simulink model "signal_based_model"  (R2025b)
settings: Solver=VariableStepAuto  StartTime=0.0  StopTime=10  RelTol=1e-3
libraries: slpidlib x4
settings Model: Creator=leo  LastModifiedBy=leo

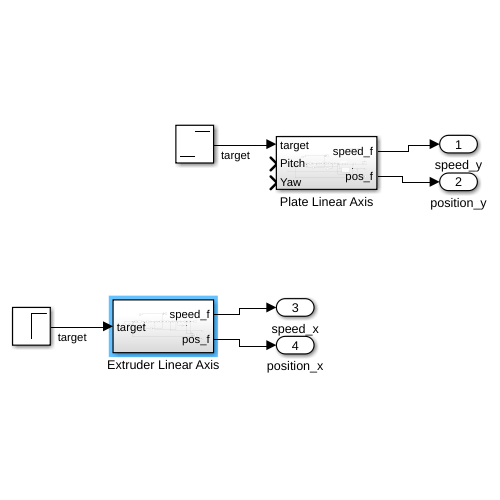
[thumbnail: Simulink's stored preview of the top-level diagram]
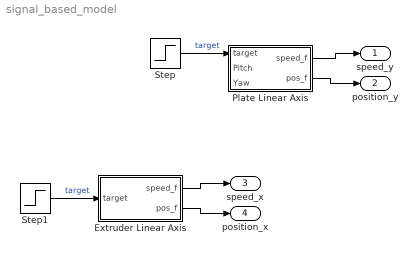
== system signal_based_model ==
  Extruder Linear Axis : Subsystem
  Plate Linear Axis : Subsystem
  Step : Step  After=0.3  SampleTime=0
  Step1 : Step  Time=0  After=0.1  SampleTime=0
  speed_y : Outport
  position_y : Outport  Port=2
  speed_x : Outport  Port=3
  position_x : Outport  Port=4
  wires:
  Step/1 -> Plate Linear Axis/1(target)  "target"
  Plate Linear Axis/1(speed_f) -> speed_y/1
  Extruder Linear Axis/2(pos_f) -> position_x/1
  Extruder Linear Axis/1(speed_f) -> speed_x/1
  Step1/1 -> Extruder Linear Axis/1(target)  "target"
  Plate Linear Axis/2(pos_f) -> position_y/1

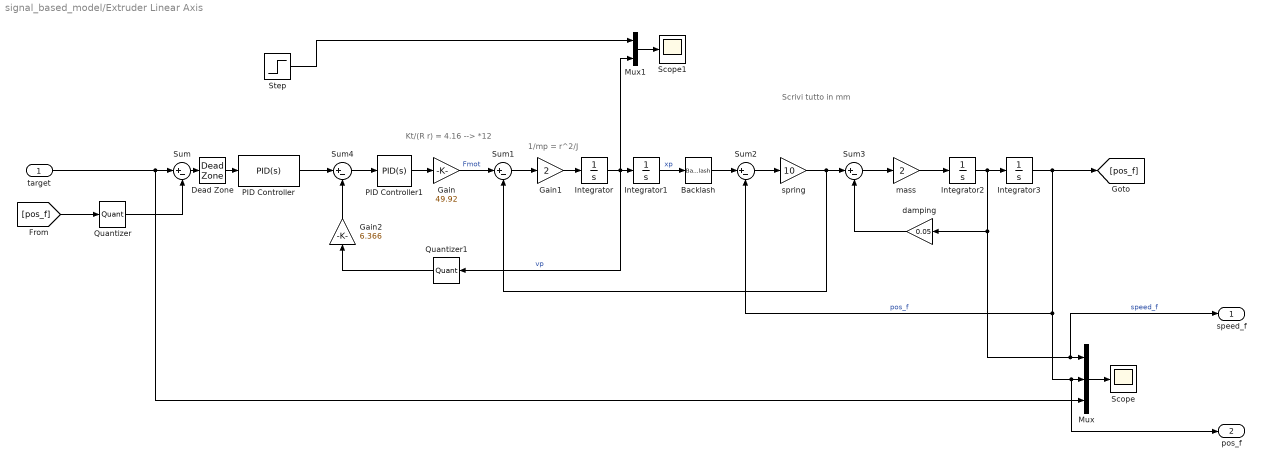
== system signal_based_model/Extruder Linear Axis ==
  note: Scrivi tutto in mm
  note: 1/mp = r^2/J
  note: Kt/(R r) = 4.16 --> *12
  target : Inport
  Backlash : Backlash  BacklashWidth=0.01
  Dead Zone : DeadZone  LowerValue=-0.005  UpperValue=0.005
  Gain : Gain  Gain=49.92
  Gain1 : Gain  Gain=2
  Gain2 : Gain  Gain=6.366
  Integrator{,1..3} (4 alike) : Integrator
  Mux : Mux  Inputs=3
  Mux1 : Mux  Inputs=2
  PID Controller : slpidlib/PID Controller  Controller=PID  Form=Parallel  TimeDomain=Continuous-time  UseExternalTs=off  SampleTime=-1  IntegratorMethod=Forward Euler  FilterMethod=Forward Euler  ControllerParametersSource=internal  P=5.88101312696394  I=1.22832421869703  UseKiTs=off  D=-1.679348597049  UseExternalDerivativeSource=off  N=2.27817359459084  UseFilter=on  TunerSelectOption=Transfer Function Based (PID Tuner App)  InitialConditionSource=internal  InitialConditionForIntegrator=0  InitialConditionForFilter=0  DifferentiatorICPrevScaledInput=0  ExternalReset=none  TrackingMode=off  Kt=1  LimitOutput=on  SatLimitsSource=internal  UpperSaturationLimit=300  LowerSaturationLimit=-300  LinearizeAsGain=on  AntiWindupMode=none  Kb=1  LimitIntegrator=off  UpperIntegratorSaturationLimit=inf  LowerIntegratorSaturationLimit=-inf  POutMin=[]  POutMax=[]  IOutMin=[]  IOutMax=[]  DOutMin=[]  DOutMax=[]  NOutMin=[]  NOutMax=[]  SumOutMin=[]  SumOutMax=[]  SaturationOutMin=[]  SaturationOutMax=[]  PParamMin=[]  PParamMax=[]  IParamMin=[]  IParamMax=[]  DParamMin=[]  DParamMax=[]  NParamMin=[]  NParamMax=[]  KbParamMin=[]  KbParamMax=[]  KtParamMin=[]  KtParamMax=[]  KbOutMin=[]  KbOutMax=[]  KtOutMin=[]  KtOutMax=[]  IntegratorOutMin=[]  IntegratorOutMax=[]  FilterOutMin=[]  FilterOutMax=[]  SumI1OutMin=[]  SumI1OutMax=[]  SumI2OutMin=[]  SumI2OutMax=[]  SumI3OutMin=[]  SumI3OutMax=[]  SumI4OutMin=[]  SumI4OutMax=[]  SumDOutMin=[]  SumDOutMax=[]  DifferentiatorOutMin=[]  DifferentiatorOutMax=[]  FilterDiffOutCoefMin=[]  FilterDiffOutCoefMax=[]  ReciprocalOutMin=[]  ReciprocalOutMax=[]  SumDenOutMin=[]  SumDenOutMax=[]  SumNumOutMin=[]  SumNumOutMax=[]  DivideOutMin=[]  DivideOutMax=[]  UdiffTsProdOutMin=[]  UdiffTsProdOutMax=[]  NTsProdOutMin=[]  NTsProdOutMax=[]  UintegralTsProdOutMin=[]  UintegralTsProdOutMax=[]  UngainTsProdOutMin=[]  UngainTsProdOutMax=[]  ClampingZeroOutDataTypeStr=Inherit: Inherit via back propagation  ClampingZeroOutMin=[]  ClampingZeroOutMax=[]  FilterDenConstantOutDataTypeStr=Inherit: Inherit via back propagation  FilterDenConstantOutMin=[]  FilterDenConstantOutMax=[]  PCopyOutDataTypeStr=Inherit: Inherit via back propagation  PCopyOutMin=[]  PCopyOutMax=[]  NCopyOutDataTypeStr=Inherit: Inherit via back propagation  NCopyOutMin=[]  NCopyOutMax=[]  IntegratorContinuousStateAttributes=''  IntegratorStateMustResolveToSignalObject=off  IntegratorRTWStateStorageClass=Auto  FilterContinuousStateAttributes=''  FilterStateMustResolveToSignalObject=off  FilterRTWStateStorageClass=Auto  ParallelPVariant=InternalParameters  IdealPVariant=Disabled  IVariant=InternalParameters  DVariant=InternalParameters  IntegratorVariant=Continuous  SatVariant=Enabled  AWVariant=Passthrough  PCopyVariant=Disabled  TRVariant=Disabled  FdbkBlocksVariant=Forward  IdealPFdbkVariant=Disabled  SatFdbkVariant=Disabled  DerivativeFilterVariant=ContFilter  NVariant=InternalParameters  NCopyVariant=Disabled  FilterICVariant=InternalICsFilter  IntegratorICVariant=InternalICs  ExternalResetVariant=Disabled  TRSumVariant=Passthrough  SumFdbkVariant=Disabled  SumVariant=Sum_PID  TsampFilterVariant=InternalTs  TsampNgainVariant=Passthrough  TsampIntegralVariant=Disabled_SignalSpec  ExternalSaturationOutDataTypeStr=Inherit: Same as second input  DerivativeSourceVariant=ErrorSignal  PreIntVariant=InternalPreInt
  PID Controller1 : slpidlib/PID Controller  Controller=PID  Form=Parallel  TimeDomain=Continuous-time  UseExternalTs=off  SampleTime=-1  IntegratorMethod=Forward Euler  FilterMethod=Forward Euler  ControllerParametersSource=internal  P=0.0150067865506817  I=0.0265065175500297  UseKiTs=off  D=0.000284995898305726  UseExternalDerivativeSource=off  N=36.46824066771  UseFilter=on  TunerSelectOption=Transfer Function Based (PID Tuner App)  InitialConditionSource=internal  InitialConditionForIntegrator=0  InitialConditionForFilter=0  DifferentiatorICPrevScaledInput=0  ExternalReset=none  TrackingMode=off  Kt=1  LimitOutput=on  SatLimitsSource=internal  UpperSaturationLimit=1  LowerSaturationLimit=-1  LinearizeAsGain=on  AntiWindupMode=none  Kb=1  LimitIntegrator=off  UpperIntegratorSaturationLimit=inf  LowerIntegratorSaturationLimit=-inf  POutMin=[]  POutMax=[]  IOutMin=[]  IOutMax=[]  DOutMin=[]  DOutMax=[]  NOutMin=[]  NOutMax=[]  SumOutMin=[]  SumOutMax=[]  SaturationOutMin=[]  SaturationOutMax=[]  PParamMin=[]  PParamMax=[]  IParamMin=[]  IParamMax=[]  DParamMin=[]  DParamMax=[]  NParamMin=[]  NParamMax=[]  KbParamMin=[]  KbParamMax=[]  KtParamMin=[]  KtParamMax=[]  KbOutMin=[]  KbOutMax=[]  KtOutMin=[]  KtOutMax=[]  IntegratorOutMin=[]  IntegratorOutMax=[]  FilterOutMin=[]  FilterOutMax=[]  SumI1OutMin=[]  SumI1OutMax=[]  SumI2OutMin=[]  SumI2OutMax=[]  SumI3OutMin=[]  SumI3OutMax=[]  SumI4OutMin=[]  SumI4OutMax=[]  SumDOutMin=[]  SumDOutMax=[]  DifferentiatorOutMin=[]  DifferentiatorOutMax=[]  FilterDiffOutCoefMin=[]  FilterDiffOutCoefMax=[]  ReciprocalOutMin=[]  ReciprocalOutMax=[]  SumDenOutMin=[]  SumDenOutMax=[]  SumNumOutMin=[]  SumNumOutMax=[]  DivideOutMin=[]  DivideOutMax=[]  UdiffTsProdOutMin=[]  UdiffTsProdOutMax=[]  NTsProdOutMin=[]  NTsProdOutMax=[]  UintegralTsProdOutMin=[]  UintegralTsProdOutMax=[]  UngainTsProdOutMin=[]  UngainTsProdOutMax=[]  ClampingZeroOutDataTypeStr=Inherit: Inherit via back propagation  ClampingZeroOutMin=[]  ClampingZeroOutMax=[]  FilterDenConstantOutDataTypeStr=Inherit: Inherit via back propagation  FilterDenConstantOutMin=[]  FilterDenConstantOutMax=[]  PCopyOutDataTypeStr=Inherit: Inherit via back propagation  PCopyOutMin=[]  PCopyOutMax=[]  NCopyOutDataTypeStr=Inherit: Inherit via back propagation  NCopyOutMin=[]  NCopyOutMax=[]  IntegratorContinuousStateAttributes=''  IntegratorStateMustResolveToSignalObject=off  IntegratorRTWStateStorageClass=Auto  FilterContinuousStateAttributes=''  FilterStateMustResolveToSignalObject=off  FilterRTWStateStorageClass=Auto  ParallelPVariant=InternalParameters  IdealPVariant=Disabled  IVariant=InternalParameters  DVariant=InternalParameters  IntegratorVariant=Continuous  SatVariant=Enabled  AWVariant=Passthrough  PCopyVariant=Disabled  TRVariant=Disabled  FdbkBlocksVariant=Forward  IdealPFdbkVariant=Disabled  SatFdbkVariant=Disabled  DerivativeFilterVariant=ContFilter  NVariant=InternalParameters  NCopyVariant=Disabled  FilterICVariant=InternalICsFilter  IntegratorICVariant=InternalICs  ExternalResetVariant=Disabled  TRSumVariant=Passthrough  SumFdbkVariant=Disabled  SumVariant=Sum_PID  TsampFilterVariant=InternalTs  TsampNgainVariant=Passthrough  TsampIntegralVariant=Disabled_SignalSpec  ExternalSaturationOutDataTypeStr=Inherit: Same as second input  DerivativeSourceVariant=ErrorSignal  PreIntVariant=InternalPreInt
  Quantizer : Quantizer  QuantizationInterval=0.005
  Quantizer1 : Quantizer  QuantizationInterval=0.02
  Scope : Scope
      settings: ActiveDisplayYMinimum=-0.12448091538103732  ActiveDisplayYMaximum=0.19087454091258427
  Scope1 : Scope
      settings: ActiveDisplayYMinimum=-1  ActiveDisplayYMaximum=1
  Step : Step  After=250  SampleTime=0
  Sum{,1..4} (5 alike) : Sum  Inputs=|+-
  damping : Gain  Gain=0.05
  mass : Gain  Gain=2
  spring : Gain  Gain=10
  speed_f : Outport
  pos_f : Outport  Port=2
  wires:
  Integrator/1 -> Mux1/2, Quantizer1/1, Integrator1/1  "vp"
  Integrator1/1 -> Backlash/1  "xp"
  Integrator3/1 -> [pos_f], Sum2/2, pos_f/1, Mux/2  "pos_f"
  Integrator2/1 -> speed_f/1, Mux/1, damping/1, Integrator3/1  "speed_f"
  Gain/1 -> Sum1/1  "Fmot"
  Gain1/1 -> Integrator/1
  Sum3/1 -> mass/1
  damping/1 -> Sum3/2
  spring/1 -> Sum1/2, Sum3/1
  Mux/1 -> Scope/1
  Sum1/1 -> Gain1/1
  Sum2/1 -> spring/1
  mass/1 -> Integrator2/1
  target/1 -> Mux/3, Sum/1
  [pos_f] -> Quantizer/1
  Backlash/1 -> Sum2/1
  Sum/1 -> Dead Zone/1
  Dead Zone/1 -> PID Controller/1
  PID Controller1/1 -> Gain/1
  Sum4/1 -> PID Controller1/1
  Quantizer1/1 -> Gain2/1
  Step/1 -> Mux1/1
  Mux1/1 -> Scope1/1
  Quantizer/1 -> Sum/2
  Gain2/1 -> Sum4/2
  PID Controller/1 -> Sum4/1

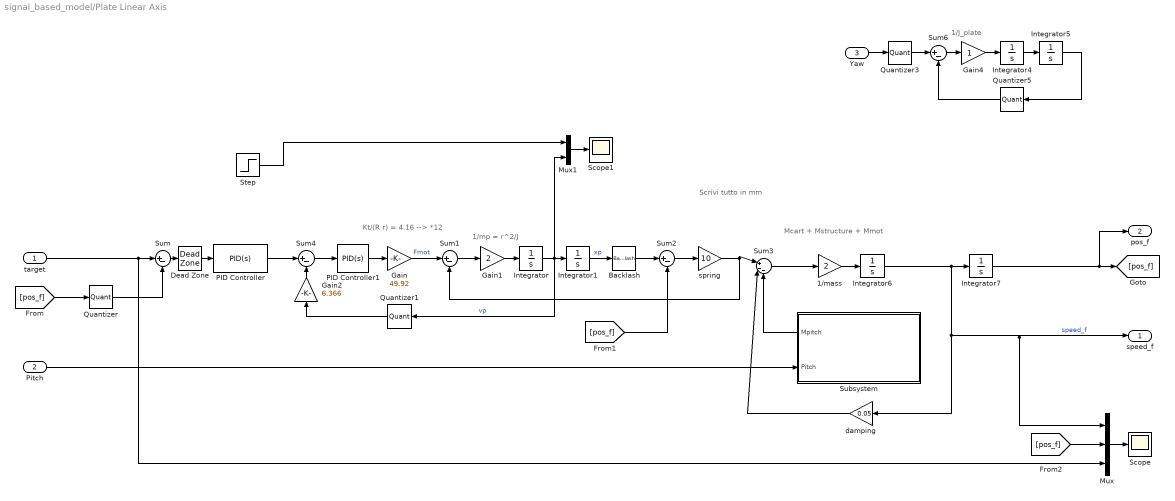
== system signal_based_model/Plate Linear Axis ==
  note: Scrivi tutto in mm
  note: 1/mp = r^2/J
  note: Kt/(R r) = 4.16 --> *12
  note: 1/J_plate
  note: Mcart + Mstructure + Mmot
  target : Inport
  Pitch : Inport  Port=2
  Yaw : Inport  Port=3
  1/mass : Gain  Gain=2
  Backlash : Backlash  BacklashWidth=0.01
  Dead Zone : DeadZone  LowerValue=-0.005  UpperValue=0.005
  Gain : Gain  Gain=49.92
  Gain1 : Gain  Gain=2
  Gain2 : Gain  Gain=6.366
  Gain4 : Gain
  Integrator{,1,4..7} (6 alike) : Integrator
  Mux : Mux  Inputs=3
  Mux1 : Mux  Inputs=2
  PID Controller : slpidlib/PID Controller  Controller=PID  Form=Parallel  TimeDomain=Continuous-time  UseExternalTs=off  SampleTime=-1  IntegratorMethod=Forward Euler  FilterMethod=Forward Euler  ControllerParametersSource=internal  P=3.73662295792307  I=0.466470585672945  UseKiTs=off  D=-1.58456449848514  UseExternalDerivativeSource=off  N=2.35813875768094  UseFilter=on  TunerSelectOption=Transfer Function Based (PID Tuner App)  InitialConditionSource=internal  InitialConditionForIntegrator=0  InitialConditionForFilter=0  DifferentiatorICPrevScaledInput=0  ExternalReset=none  TrackingMode=off  Kt=1  LimitOutput=on  SatLimitsSource=internal  UpperSaturationLimit=300  LowerSaturationLimit=-300  LinearizeAsGain=on  AntiWindupMode=none  Kb=1  LimitIntegrator=off  UpperIntegratorSaturationLimit=inf  LowerIntegratorSaturationLimit=-inf  POutMin=[]  POutMax=[]  IOutMin=[]  IOutMax=[]  DOutMin=[]  DOutMax=[]  NOutMin=[]  NOutMax=[]  SumOutMin=[]  SumOutMax=[]  SaturationOutMin=[]  SaturationOutMax=[]  PParamMin=[]  PParamMax=[]  IParamMin=[]  IParamMax=[]  DParamMin=[]  DParamMax=[]  NParamMin=[]  NParamMax=[]  KbParamMin=[]  KbParamMax=[]  KtParamMin=[]  KtParamMax=[]  KbOutMin=[]  KbOutMax=[]  KtOutMin=[]  KtOutMax=[]  IntegratorOutMin=[]  IntegratorOutMax=[]  FilterOutMin=[]  FilterOutMax=[]  SumI1OutMin=[]  SumI1OutMax=[]  SumI2OutMin=[]  SumI2OutMax=[]  SumI3OutMin=[]  SumI3OutMax=[]  SumI4OutMin=[]  SumI4OutMax=[]  SumDOutMin=[]  SumDOutMax=[]  DifferentiatorOutMin=[]  DifferentiatorOutMax=[]  FilterDiffOutCoefMin=[]  FilterDiffOutCoefMax=[]  ReciprocalOutMin=[]  ReciprocalOutMax=[]  SumDenOutMin=[]  SumDenOutMax=[]  SumNumOutMin=[]  SumNumOutMax=[]  DivideOutMin=[]  DivideOutMax=[]  UdiffTsProdOutMin=[]  UdiffTsProdOutMax=[]  NTsProdOutMin=[]  NTsProdOutMax=[]  UintegralTsProdOutMin=[]  UintegralTsProdOutMax=[]  UngainTsProdOutMin=[]  UngainTsProdOutMax=[]  ClampingZeroOutDataTypeStr=Inherit: Inherit via back propagation  ClampingZeroOutMin=[]  ClampingZeroOutMax=[]  FilterDenConstantOutDataTypeStr=Inherit: Inherit via back propagation  FilterDenConstantOutMin=[]  FilterDenConstantOutMax=[]  PCopyOutDataTypeStr=Inherit: Inherit via back propagation  PCopyOutMin=[]  PCopyOutMax=[]  NCopyOutDataTypeStr=Inherit: Inherit via back propagation  NCopyOutMin=[]  NCopyOutMax=[]  IntegratorContinuousStateAttributes=''  IntegratorStateMustResolveToSignalObject=off  IntegratorRTWStateStorageClass=Auto  FilterContinuousStateAttributes=''  FilterStateMustResolveToSignalObject=off  FilterRTWStateStorageClass=Auto  ParallelPVariant=InternalParameters  IdealPVariant=Disabled  IVariant=InternalParameters  DVariant=InternalParameters  IntegratorVariant=Continuous  SatVariant=Enabled  AWVariant=Passthrough  PCopyVariant=Disabled  TRVariant=Disabled  FdbkBlocksVariant=Forward  IdealPFdbkVariant=Disabled  SatFdbkVariant=Disabled  DerivativeFilterVariant=ContFilter  NVariant=InternalParameters  NCopyVariant=Disabled  FilterICVariant=InternalICsFilter  IntegratorICVariant=InternalICs  ExternalResetVariant=Disabled  TRSumVariant=Passthrough  SumFdbkVariant=Disabled  SumVariant=Sum_PID  TsampFilterVariant=InternalTs  TsampNgainVariant=Passthrough  TsampIntegralVariant=Disabled_SignalSpec  ExternalSaturationOutDataTypeStr=Inherit: Same as second input  DerivativeSourceVariant=ErrorSignal  PreIntVariant=InternalPreInt
  PID Controller1 : slpidlib/PID Controller  Controller=PID  Form=Parallel  TimeDomain=Continuous-time  UseExternalTs=off  SampleTime=-1  IntegratorMethod=Forward Euler  FilterMethod=Forward Euler  ControllerParametersSource=internal  P=0.0150067865506817  I=0.0265065175500297  UseKiTs=off  D=0.000284995898305726  UseExternalDerivativeSource=off  N=36.46824066771  UseFilter=on  TunerSelectOption=Transfer Function Based (PID Tuner App)  InitialConditionSource=internal  InitialConditionForIntegrator=0  InitialConditionForFilter=0  DifferentiatorICPrevScaledInput=0  ExternalReset=none  TrackingMode=off  Kt=1  LimitOutput=on  SatLimitsSource=internal  UpperSaturationLimit=1  LowerSaturationLimit=-1  LinearizeAsGain=on  AntiWindupMode=none  Kb=1  LimitIntegrator=off  UpperIntegratorSaturationLimit=inf  LowerIntegratorSaturationLimit=-inf  POutMin=[]  POutMax=[]  IOutMin=[]  IOutMax=[]  DOutMin=[]  DOutMax=[]  NOutMin=[]  NOutMax=[]  SumOutMin=[]  SumOutMax=[]  SaturationOutMin=[]  SaturationOutMax=[]  PParamMin=[]  PParamMax=[]  IParamMin=[]  IParamMax=[]  DParamMin=[]  DParamMax=[]  NParamMin=[]  NParamMax=[]  KbParamMin=[]  KbParamMax=[]  KtParamMin=[]  KtParamMax=[]  KbOutMin=[]  KbOutMax=[]  KtOutMin=[]  KtOutMax=[]  IntegratorOutMin=[]  IntegratorOutMax=[]  FilterOutMin=[]  FilterOutMax=[]  SumI1OutMin=[]  SumI1OutMax=[]  SumI2OutMin=[]  SumI2OutMax=[]  SumI3OutMin=[]  SumI3OutMax=[]  SumI4OutMin=[]  SumI4OutMax=[]  SumDOutMin=[]  SumDOutMax=[]  DifferentiatorOutMin=[]  DifferentiatorOutMax=[]  FilterDiffOutCoefMin=[]  FilterDiffOutCoefMax=[]  ReciprocalOutMin=[]  ReciprocalOutMax=[]  SumDenOutMin=[]  SumDenOutMax=[]  SumNumOutMin=[]  SumNumOutMax=[]  DivideOutMin=[]  DivideOutMax=[]  UdiffTsProdOutMin=[]  UdiffTsProdOutMax=[]  NTsProdOutMin=[]  NTsProdOutMax=[]  UintegralTsProdOutMin=[]  UintegralTsProdOutMax=[]  UngainTsProdOutMin=[]  UngainTsProdOutMax=[]  ClampingZeroOutDataTypeStr=Inherit: Inherit via back propagation  ClampingZeroOutMin=[]  ClampingZeroOutMax=[]  FilterDenConstantOutDataTypeStr=Inherit: Inherit via back propagation  FilterDenConstantOutMin=[]  FilterDenConstantOutMax=[]  PCopyOutDataTypeStr=Inherit: Inherit via back propagation  PCopyOutMin=[]  PCopyOutMax=[]  NCopyOutDataTypeStr=Inherit: Inherit via back propagation  NCopyOutMin=[]  NCopyOutMax=[]  IntegratorContinuousStateAttributes=''  IntegratorStateMustResolveToSignalObject=off  IntegratorRTWStateStorageClass=Auto  FilterContinuousStateAttributes=''  FilterStateMustResolveToSignalObject=off  FilterRTWStateStorageClass=Auto  ParallelPVariant=InternalParameters  IdealPVariant=Disabled  IVariant=InternalParameters  DVariant=InternalParameters  IntegratorVariant=Continuous  SatVariant=Enabled  AWVariant=Passthrough  PCopyVariant=Disabled  TRVariant=Disabled  FdbkBlocksVariant=Forward  IdealPFdbkVariant=Disabled  SatFdbkVariant=Disabled  DerivativeFilterVariant=ContFilter  NVariant=InternalParameters  NCopyVariant=Disabled  FilterICVariant=InternalICsFilter  IntegratorICVariant=InternalICs  ExternalResetVariant=Disabled  TRSumVariant=Passthrough  SumFdbkVariant=Disabled  SumVariant=Sum_PID  TsampFilterVariant=InternalTs  TsampNgainVariant=Passthrough  TsampIntegralVariant=Disabled_SignalSpec  ExternalSaturationOutDataTypeStr=Inherit: Same as second input  DerivativeSourceVariant=ErrorSignal  PreIntVariant=InternalPreInt
  Quantizer : Quantizer  QuantizationInterval=0.01
  Quantizer1 : Quantizer  QuantizationInterval=0.02
  Quantizer3 : Quantizer
  Quantizer5 : Quantizer
  Scope : Scope
      settings: ActiveDisplayYMinimum=-1.0744185087165565  ActiveDisplayYMaximum=1.0049223218652417
  Scope1 : Scope
      settings: ActiveDisplayYMinimum=-1  ActiveDisplayYMaximum=1
  Step : Step  After=250  SampleTime=0
  Subsystem : Subsystem
      settings: PortSchema="{\"entries\":[{\"content\":{\"sides\":[{\"content\":{\"connectorIds\":[\"Out1\",\"In1\"]},\"type\":\"ConnectorPlacement.EquallySpacedRectSide\",\"uuid\":\"c6fbe630-3349-497f-9dd7-90e0f83e84b9\"},{\"content\":{\"side\":\"RIGHT\"},\"type\":\"ConnectorPlacement.EquallySpacedRectSide\",\"uuid\":\"ffa0a2d0-f213-47a0-84af-10fed00c1f85\"},{\"content\":{\"side\":\"TOP\"},\"type\":\"ConnectorPlacement.EquallySpacedRectSide\",\"uuid\":\"5dd9fa2b-7a91-4dc9-91b0-f07acfc95730\"}]},\"type\":\"ConnectorPlacement.EquallySpacedConnector\",\"uuid\":\"75913121-a205-499e-a3df-ddb329c0f5be\"}],\"packageUris\":[\"http://schema.mathworks.com/mf0/Connector/R2020b\"],\"version\":\"1.0\"}"
  Sum{,1..2,4,6} (5 alike) : Sum  Inputs=|+-
  Sum3 : Sum  Inputs=|+--
  damping : Gain  Gain=0.05
  spring : Gain  Gain=10
  speed_f : Outport
  pos_f : Outport  Port=2
  wires:
  Integrator/1 -> Mux1/2, Quantizer1/1, Integrator1/1  "vp"
  Integrator1/1 -> Backlash/1  "xp"
  Gain/1 -> Sum1/1  "Fmot"
  Gain1/1 -> Integrator/1
  spring/1 -> Sum1/2, Sum3/1
  Mux/1 -> Scope/1
  Sum1/1 -> Gain1/1
  Sum2/1 -> spring/1
  target/1 -> Mux/3, Sum/1
  [pos_f] -> Quantizer/1
  Backlash/1 -> Sum2/1
  Sum/1 -> Dead Zone/1
  Dead Zone/1 -> PID Controller/1
  PID Controller1/1 -> Gain/1
  Sum4/1 -> PID Controller1/1
  Quantizer1/1 -> Gain2/1
  Step/1 -> Mux1/1
  Mux1/1 -> Scope1/1
  Quantizer/1 -> Sum/2
  Gain2/1 -> Sum4/2
  PID Controller/1 -> Sum4/1
  Integrator7/1 -> pos_f/1, [pos_f]
  Sum3/1 -> 1/mass/1
  Sum6/1 -> Gain4/1
  Quantizer5/1 -> Sum6/2
  Quantizer3/1 -> Sum6/1
  Gain4/1 -> Integrator4/1
  Integrator5/1 -> Quantizer5/1
  Integrator4/1 -> Integrator5/1
  Yaw/1 -> Quantizer3/1
  Integrator6/1 -> damping/1, Mux/1, speed_f/1, Integrator7/1  "speed_f"
  1/mass/1 -> Integrator6/1
  damping/1 -> Sum3/2
  Pitch/1 -> Subsystem/1(Pitch)
  Subsystem/1(Mpitch) -> Sum3/3
  [pos_f] -> Mux/2
  [pos_f] -> Sum2/2

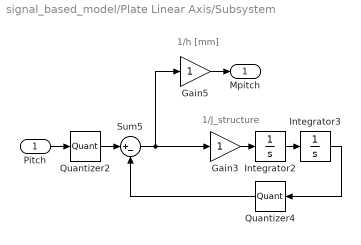
== system signal_based_model/Plate Linear Axis/Subsystem ==
  note: 1/h [mm]
  note: 1/J_structure
  Pitch : Inport
  Gain3 : Gain
  Gain5 : Gain
  Integrator2 : Integrator
  Integrator3 : Integrator
  Quantizer2 : Quantizer
  Quantizer4 : Quantizer
  Sum5 : Sum  Inputs=|+-
  Mpitch : Outport
  wires:
  Integrator3/1 -> Quantizer4/1
  Pitch/1 -> Quantizer2/1
  Integrator2/1 -> Integrator3/1
  Sum5/1 -> Gain5/1, Gain3/1
  Quantizer2/1 -> Sum5/1
  Gain3/1 -> Integrator2/1
  Quantizer4/1 -> Sum5/2
  Gain5/1 -> Mpitch/1
